simulink model "lab8"  (R2025b)
settings: Solver=VariableStepAuto  StartTime=0.0  StopTime=10.0  MaxStep=0.01  RelTol=1e-6  AbsTol=1e-8
undefined symbols (not defined in the file): a0, bmin, gamma2, sgn, task2
settings Model: Creator=Nickolay  LastModifiedBy=Nickolay

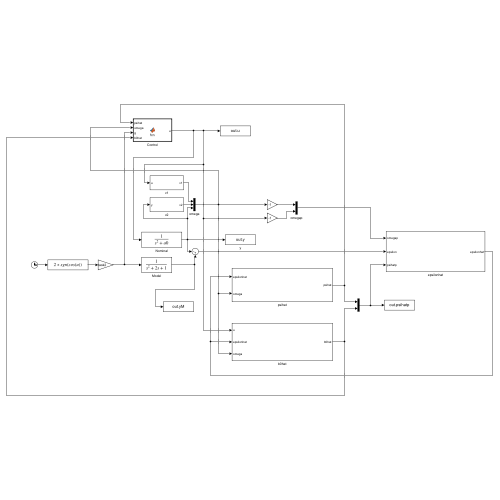
[thumbnail: Simulink's stored preview of the top-level diagram]
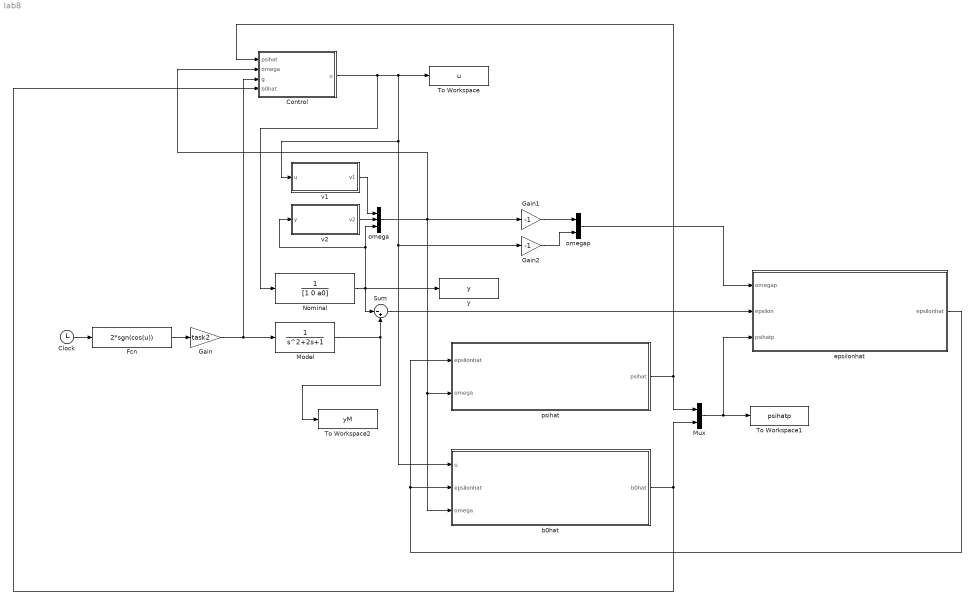
== system lab8 ==
  Clock : Clock
  Control : MATLAB Function  TreatAsAtomicUnit=on
  Fcn : Fcn  Expr=2*sgn(cos(u))
  Gain : Gain  Gain=task2
  Gain1 : Gain  Gain=-1
  Gain2 : Gain  Gain=-1
  Model : TransferFcn
  Mux : Mux  Inputs=2
  Nominal : TransferFcn  Denominator=[1 0 a0]
  Sum : Sum  Inputs=|-+
  To Workspace : ToWorkspace  VariableName=u  SaveFormat=Timeseries  SampleTime=-1
  To Workspace1 : ToWorkspace  VariableName=psihatp  SaveFormat=Timeseries  SampleTime=-1
  To Workspace2 : ToWorkspace  VariableName=yM  SaveFormat=Timeseries  SampleTime=-1
  b0hat : Subsystem
  epsilonhat : Subsystem
  omega : Mux  Inputs=3
  omegap : Mux  Inputs=2
  psihat : Subsystem
  v1 : Subsystem
  v2 : Subsystem
  y : ToWorkspace  VariableName=y  SaveFormat=Timeseries  SampleTime=-1
  wires:
  Fcn/1 -> Gain/1
  Clock/1 -> Fcn/1
  Gain/1 -> Model/1, Control/3(g)
  epsilonhat/1(epsilonhat) -> psihat/1(epsilonhat), b0hat/2(epsilonhat)
  psihat/1(psihat) -> Control/1(psihat), Mux/1
  b0hat/1(b0hat) -> Mux/2, Control/4(b0hat)
  Mux/1 -> To Workspace1/1, epsilonhat/3(psihatp)
  v1/1(v1) -> omega/1
  v2/1(v2) -> omega/2
  Nominal/1 -> omega/3, v2/1(y), y/1, Sum/1
  omega/1 -> Gain1/1, psihat/2(omega), b0hat/3(omega), Control/2(omega)
  Gain1/1 -> omegap/1
  Gain2/1 -> omegap/2
  omegap/1 -> epsilonhat/1(omegap)
  Sum/1 -> epsilonhat/2(epsilon)
  Control/1(u) -> To Workspace/1, b0hat/1(u), Gain2/1, v1/1(u), Nominal/1
  Model/1 -> To Workspace2/1, Sum/2

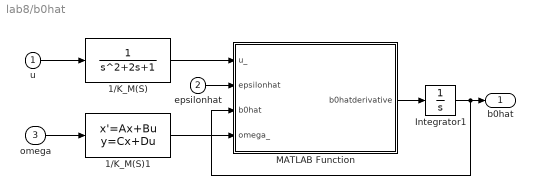
== system lab8/b0hat ==
  u : Inport
  epsilonhat : Inport  Port=2
  omega : Inport  Port=3
  1/K_M(S) : TransferFcn
  1/K_M(S)1 : StateSpace  A=kron(eye(3),[0 1;-1 -2])  B=kron(eye(3),[0;1])  C=kron(eye(3),[1 0])  D=zeros(3)  InitialCondition=0
  Integrator1 : Integrator  InitialCondition=2
  MATLAB Function : MATLAB Function  TreatAsAtomicUnit=on
  b0hat : Outport
  wires:
  epsilonhat/1 -> MATLAB Function/2(epsilonhat)
  MATLAB Function/1(b0hatderivative) -> Integrator1/1
  Integrator1/1 -> MATLAB Function/3(b0hat), b0hat/1
  1/K_M(S)/1 -> MATLAB Function/1(u_)
  u/1 -> 1/K_M(S)/1
  1/K_M(S)1/1 -> MATLAB Function/4(omega_)
  omega/1 -> 1/K_M(S)1/1

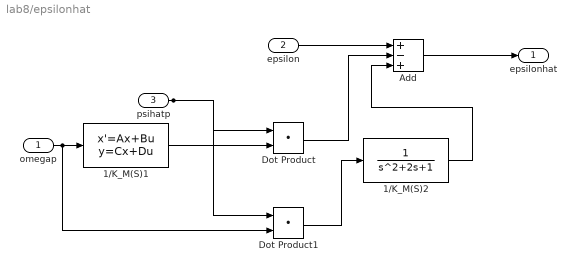
== system lab8/epsilonhat ==
  omegap : Inport
  epsilon : Inport  Port=2
  psihatp : Inport  Port=3
  1/K_M(S)1 : StateSpace  A=kron(eye(4),[0 1;-1 -2])  B=kron(eye(4),[0;1])  C=kron(eye(4),[1 0])  D=zeros(4)  InitialCondition=0
  1/K_M(S)2 : TransferFcn
  Add : Sum  Inputs=+-+
  Dot Product : DotProduct  OutDataTypeStr=Inherit: Inherit via internal rule
  Dot Product1 : DotProduct  OutDataTypeStr=Inherit: Inherit via internal rule
  epsilonhat : Outport
  wires:
  epsilon/1 -> Add/1
  Add/1 -> epsilonhat/1
  omegap/1 -> Dot Product1/2, 1/K_M(S)1/1
  1/K_M(S)1/1 -> Dot Product/2
  Dot Product/1 -> Add/2
  Dot Product1/1 -> 1/K_M(S)2/1
  1/K_M(S)2/1 -> Add/3
  psihatp/1 -> Dot Product/1, Dot Product1/1

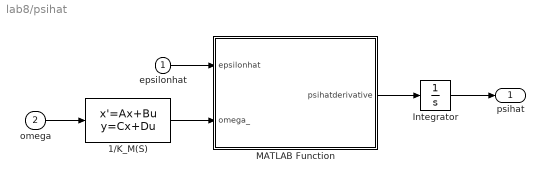
== system lab8/psihat ==
  epsilonhat : Inport
  omega : Inport  Port=2
  1/K_M(S) : StateSpace  A=kron(eye(3),[0 1;-1 -2])  B=kron(eye(3),[0;1])  C=kron(eye(3),[1 0])  D=zeros(3)  InitialCondition=0
  Integrator : Integrator  InitialCondition=[1;1;1]
  MATLAB Function : MATLAB Function  TreatAsAtomicUnit=on
  psihat : Outport
  wires:
  Integrator/1 -> psihat/1
  omega/1 -> 1/K_M(S)/1
  1/K_M(S)/1 -> MATLAB Function/2(omega_)
  epsilonhat/1 -> MATLAB Function/1(epsilonhat)
  MATLAB Function/1(psihatderivative) -> Integrator/1

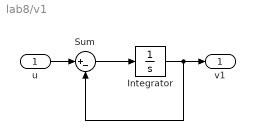
== system lab8/v1 ==
  u : Inport
  Integrator : Integrator  InitialCondition=1
  Sum : Sum  Inputs=|+-
  v1 : Outport
  wires:
  Integrator/1 -> Sum/2, v1/1
  u/1 -> Sum/1
  Sum/1 -> Integrator/1

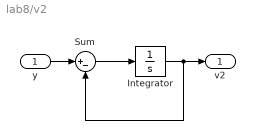
== system lab8/v2 ==
  y : Inport
  Integrator : Integrator  InitialCondition=1
  Sum : Sum  Inputs=|+-
  v2 : Outport
  wires:
  Integrator/1 -> Sum/2, v2/1
  y/1 -> Sum/1
  Sum/1 -> Integrator/1

== matlab function lab8/psihat/MATLAB Function ==
  data: epsilonhat input; omega_ input; psihatderivative output; gamma1 parameter
function psihatderivative  = fcn(epsilonhat, omega_, gamma1)

psihatderivative  = -gamma1 * omega_ * epsilonhat / (1 + omega_.' * omega_);

end

== matlab function lab8/b0hat/MATLAB Function ==
  data: u_ input; b0hatderivative output; epsilonhat input; b0hat input; omega_ input; bmin parameter; gamma2 parameter
function b0hatderivative = fcn(u_, epsilonhat, b0hat, omega_, bmin, gamma2)

q = -gamma2 * u_ * epsilonhat / (1 + omega_.' * omega_);

if b0hat >= bmin
    b0hatderivative = q;
else
    b0hatderivative = 0;
end

end

== matlab function lab8/Control ==
  data: psihat input; u output; omega input; g input; b0hat input
function u = fcn(psihat, omega, g, b0hat)
u = (g-psihat.'*omega)/b0hat;
